simulink model "lab_1_3"  (R2023b)
settings: Solver=FixedStepAuto  StartTime=0.0  StopTime=10.0  FixedStep=0.001  RelTol=1e-3
settings Model: Creator=nsukh  LastModifiedBy=nsukh

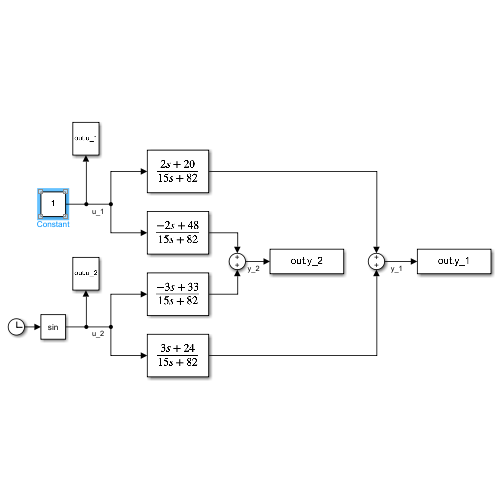
[thumbnail: Simulink's stored preview of the top-level diagram]
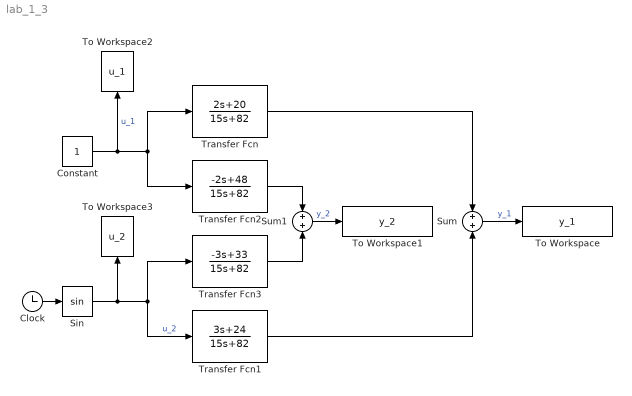
== system lab_1_3 ==
  Clock : Clock
  Constant : Constant  SampleTime=-1
  Sin : Trigonometry
  Sum : Sum  Inputs=+|+
  Sum1 : Sum  Inputs=+|+
  To Workspace : ToWorkspace  VariableName=y_1  SaveFormat=Timeseries  SampleTime=-1
  To Workspace1 : ToWorkspace  VariableName=y_2  SaveFormat=Timeseries  SampleTime=-1
  To Workspace2 : ToWorkspace  VariableName=u_1  SaveFormat=Timeseries  SampleTime=-1
  To Workspace3 : ToWorkspace  VariableName=u_2  SaveFormat=Timeseries  SampleTime=-1
  Transfer Fcn : TransferFcn  Numerator=[2 20]  Denominator=[15 82]
  Transfer Fcn1 : TransferFcn  Numerator=[3 24]  Denominator=[15 82]
  Transfer Fcn2 : TransferFcn  Numerator=[-2 48]  Denominator=[15 82]
  Transfer Fcn3 : TransferFcn  Numerator=[-3 33]  Denominator=[15 82]
  wires:
  Clock/1 -> Sin/1
  Constant/1 -> To Workspace2/1, Transfer Fcn2/1, Transfer Fcn/1  "u_1"
  Sin/1 -> To Workspace3/1, Transfer Fcn3/1, Transfer Fcn1/1  "u_2"
  Transfer Fcn/1 -> Sum/1
  Sum/1 -> To Workspace/1  "y_1"
  Transfer Fcn1/1 -> Sum/2
  Transfer Fcn2/1 -> Sum1/1
  Transfer Fcn3/1 -> Sum1/2
  Sum1/1 -> To Workspace1/1  "y_2"
